simulink model "M1_FirstPrinciplesMotor"  (R2026a)
settings: Solver=ode15s  StopTime=2  MaxStep=0.001
settings Model: Creator=siddh  LastModifiedBy=sjawahar

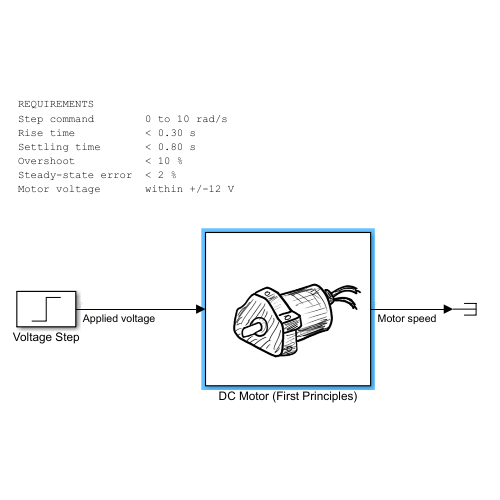
[thumbnail: Simulink's stored preview of the top-level diagram]
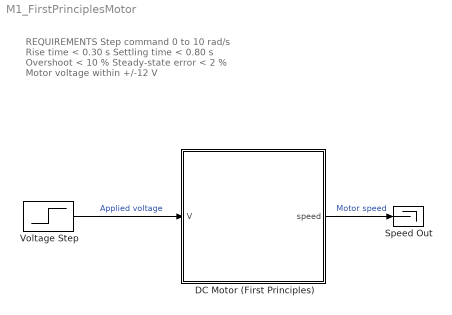
== system M1_FirstPrinciplesMotor ==
  note: REQUIREMENTS
      | Step command        0 to 10 rad/s
      | Rise time           < 0.30 s
      | Settling time       < 0.80 s
      | Overshoot           < 10 %
      | Steady-state error  < 2 %
      | Motor voltage       within +/-12 V
  DC Motor (First Principles) : Subsystem
      mask Display: image('DC motor.png')
  Speed Out : Terminator
  Voltage Step : Step  Time=0.1  FinalValue=2  SampleTime=0
  wires:
  Voltage Step/1 -> DC Motor (First Principles)/1(V)  "Applied voltage"
  DC Motor (First Principles)/1(speed) -> Speed Out/1  "Motor speed"

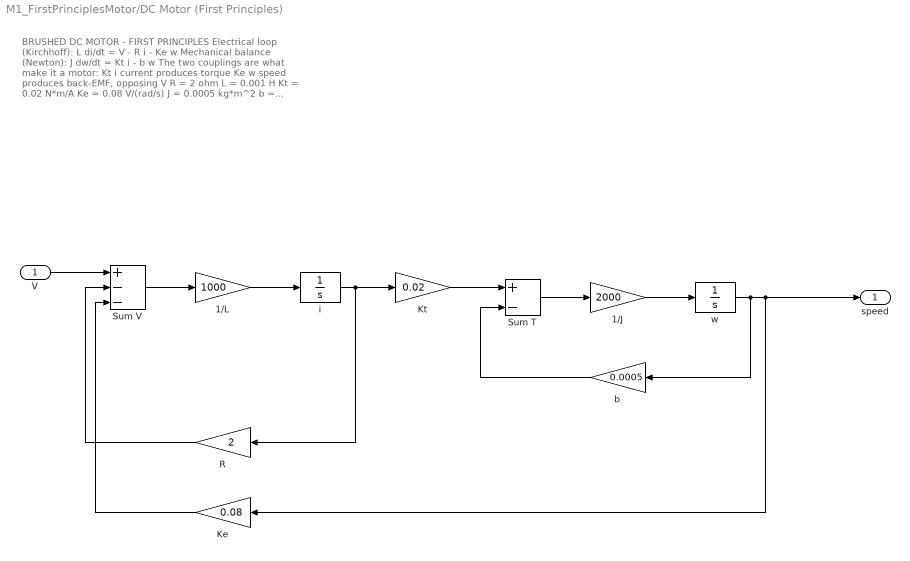
== system M1_FirstPrinciplesMotor/DC Motor (First Principles) ==
  note: BRUSHED DC MOTOR - FIRST PRINCIPLES
      |
      | Electrical loop (Kirchhoff):
      |     L di/dt = V - R i - Ke w
      |
      | Mechanical balance (Newton):
      |     J dw/dt = Kt i - b w
      |
      | The two couplings are what make it a motor:
      |     Kt i    current produces torque
      |     Ke w    speed produces back-EMF, opposing V
      |
      | R  = 2 ohm        L  = 0.001 H
      | Kt = 0.02 N*m/A    Ke = 0.08 V/(rad/s)
      | J  = 0.0005 kg*m^2   b  = 0.0005 N*m/(rad/s)
  V : Inport
  1/J : Gain  Gain=2000
  1/L : Gain  Gain=1000
  Ke : Gain  Gain=0.08
  Kt : Gain  Gain=0.02
  R : Gain  Gain=2
  Sum T : Sum  Inputs=+-
  Sum V : Sum  Inputs=+--
  b : Gain  Gain=0.0005
  i : Integrator
  w : Integrator
  speed : Outport
  wires:
  V/1 -> Sum V/1
  Sum V/1 -> 1/L/1
  1/L/1 -> i/1
  i/1 -> Kt/1, R/1
  Kt/1 -> Sum T/1
  Sum T/1 -> 1/J/1
  1/J/1 -> w/1
  w/1 -> speed/1, Ke/1, b/1
  b/1 -> Sum T/2
  R/1 -> Sum V/2
  Ke/1 -> Sum V/3
